simulink model "XMECH01_reference"  (R2025a)
settings: Solver=FixedStepDiscrete  StartTime=0  StopTime=12  FixedStep=0.0050000000000000001  RelTol=1e-3
undefined symbols (not defined in the file): grade_angle, left_track_command, left_traction_loss, payload_mass, right_track_command, terrain_friction, traction_event_time
settings Model: Creator=SimuVerity Contributors  LastModifiedBy=SimuVerity Contributors

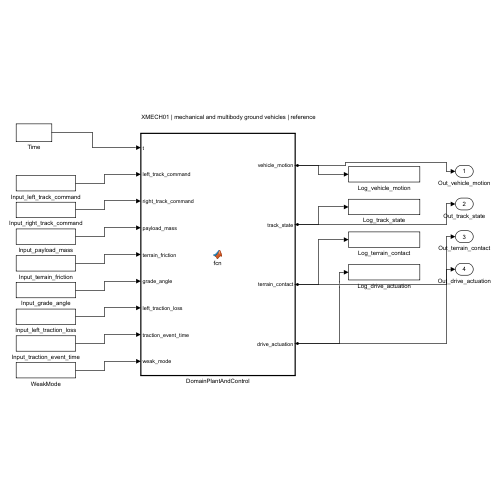
[thumbnail: Simulink's stored preview of the top-level diagram]
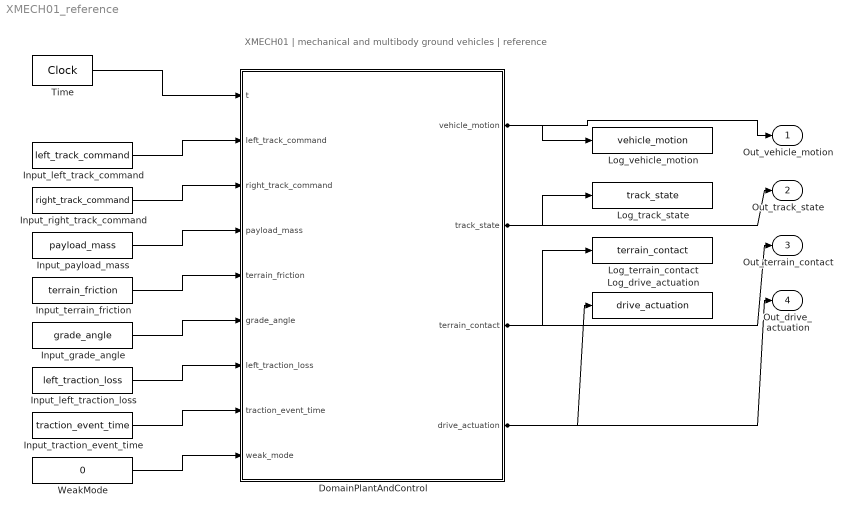
== system XMECH01_reference ==
  note: XMECH01 | mechanical and multibody ground vehicles | reference
  DomainPlantAndControl : MATLAB Function  TreatAsAtomicUnit=on
  Input_grade_angle : Constant  Value=grade_angle
  Input_left_track_command : Constant  Value=left_track_command
  Input_left_traction_loss : Constant  Value=left_traction_loss
  Input_payload_mass : Constant  Value=payload_mass
  Input_right_track_command : Constant  Value=right_track_command
  Input_terrain_friction : Constant  Value=terrain_friction
  Input_traction_event_time : Constant  Value=traction_event_time
  Log_drive_actuation : ToWorkspace  VariableName=drive_actuation  SaveFormat=Timeseries  SampleTime=-1
  Log_terrain_contact : ToWorkspace  VariableName=terrain_contact  SaveFormat=Timeseries  SampleTime=-1
  Log_track_state : ToWorkspace  VariableName=track_state  SaveFormat=Timeseries  SampleTime=-1
  Log_vehicle_motion : ToWorkspace  VariableName=vehicle_motion  SaveFormat=Timeseries  SampleTime=-1
  Time : DigitalClock  SampleTime=0.0050000000000000001
  WeakMode : Constant  Value=0
  Out_vehicle_motion : Outport
  Out_track_state : Outport  Port=2
  Out_terrain_contact : Outport  Port=3
  Out_drive_actuation : Outport  Port=4
  wires:
  Time/1 -> DomainPlantAndControl/1(t)
  Input_left_track_command/1 -> DomainPlantAndControl/2(left_track_command)
  Input_right_track_command/1 -> DomainPlantAndControl/3(right_track_command)
  Input_payload_mass/1 -> DomainPlantAndControl/4(payload_mass)
  Input_terrain_friction/1 -> DomainPlantAndControl/5(terrain_friction)
  Input_grade_angle/1 -> DomainPlantAndControl/6(grade_angle)
  Input_left_traction_loss/1 -> DomainPlantAndControl/7(left_traction_loss)
  Input_traction_event_time/1 -> DomainPlantAndControl/8(traction_event_time)
  WeakMode/1 -> DomainPlantAndControl/9(weak_mode)
  DomainPlantAndControl/1(vehicle_motion) -> Log_vehicle_motion/1, Out_vehicle_motion/1
  DomainPlantAndControl/2(track_state) -> Log_track_state/1, Out_track_state/1
  DomainPlantAndControl/3(terrain_contact) -> Log_terrain_contact/1, Out_terrain_contact/1
  DomainPlantAndControl/4(drive_actuation) -> Log_drive_actuation/1, Out_drive_actuation/1

== matlab function XMECH01_reference/DomainPlantAndControl ==
  data: t input; vehicle_motion output; left_track_command input; right_track_command input; payload_mass input; terrain_friction input; grade_angle input; left_traction_loss input; traction_event_time input; weak_mode input; track_state output; terrain_contact output; drive_actuation output
function [vehicle_motion,track_state,terrain_contact,drive_actuation] = fcn(t,left_track_command,right_track_command,payload_mass,terrain_friction,grade_angle,left_traction_loss,traction_event_time,weak_mode)
%#codegen
persistent x y psi v r uL uR iL iR
dt=0.005; g=9.81; width=1.2; m=720+payload_mass; Izz=610+0.62*payload_mass;
if isempty(x)
    x=0; y=0; psi=0; v=0; r=0; uL=0; uR=0; iL=0; iR=0;
end
grade=grade_angle*pi/180; event=(t>=traction_event_time && t<traction_event_time+1.2);
NL=0.5*m*g*cos(grade); NR=NL;
if weak_mode<0.5
    vLbody=v-0.5*width*r; vRbody=v+0.5*width*r;
    sL=uL-vLbody; sR=uR-vRbody;
    muL=terrain_friction*(1-left_traction_loss*double(event)); muR=terrain_friction;
    FL=muL*NL*tanh(3.0*sL); FR=muR*NR*tanh(3.0*sR);
    eL=left_track_command-uL; eR=right_track_command-uR;
    iL=min(max(iL+eL*dt,-2.5),2.5); iR=min(max(iR+eR*dt,-2.5),2.5);
    driveL=min(max(3900*eL+1850*iL,-7200),7200);
    driveR=min(max(3900*eR+1850*iR,-7200),7200);
    duL=(driveL-FL-95*uL)/58; duR=(driveR-FR-95*uR)/58;
    drag=105*v+34*v*abs(v);
    dv=(FL+FR-drag-m*g*sin(grade))/m;
    dr=((FR-FL)*0.5*width-420*r)/Izz;
elseif weak_mode<1.5
    duL=(left_track_command-uL)/0.16; duR=(right_track_command-uR)/0.16;
    vTarget=0.5*(left_track_command+right_track_command);
    rTarget=(right_track_command-left_track_command)/width;
    dv=(vTarget-v)/0.38; dr=(rTarget-r)/0.32;
    FL=0.5*(105*v+34*v*abs(v)+m*g*sin(grade)); FR=FL;
    driveL=FL+95*uL; driveR=FR+95*uR;
else
    % Developer shortcut mutant: prescribed chassis kinematics with
    % plausible self-reported contact and drive signals.  It is used
    % only to red-team the scorer and is never selected by the golden.
    duL=(left_track_command-uL)/0.16; duR=(right_track_command-uR)/0.16;
    vTarget=0.5*(left_track_command+right_track_command);
    rTarget=(right_track_command-left_track_command)/width;
    dv=(vTarget-v)/0.38; dr=(rTarget-r)/0.32;
    fakeLoss=left_traction_loss*double(event);
    baseF=0.5*(105*v+34*v*abs(v)+m*g*sin(grade));
    FL=baseF*(1-0.45*fakeLoss); FR=baseF*(1+0.15*fakeLoss);
    driveL=FL+58*duL+95*uL; driveR=FR+58*duR+95*uR;
end
uL=uL+dt*duL; uR=uR+dt*duR; v=v+dt*dv; r=r+dt*dr;
psi=psi+dt*r; x=x+dt*v*cos(psi); y=y+dt*v*sin(psi);
vLbody=v-0.5*width*r; vRbody=v+0.5*width*r;
slipL=(uL-vLbody)/max(max(abs(uL),abs(vLbody)),0.35); slipR=(uR-vRbody)/max(max(abs(uR),abs(vRbody)),0.35);
if weak_mode>=1.5,slipL=slipL+0.18*left_traction_loss*double(event);end
vehicle_motion=[x,y,psi,v,r];
track_state=[uL,uR,slipL,slipR];
terrain_contact=[FL,FR,NL,NR];
drive_actuation=[driveL,driveR];
end
